simulink model "pgfm_droop"  (R2026b)
settings: Solver=ode1  StartTime=0  StopTime=param.tb.t_end  FixedStep=param.sim.tc
values from neighbouring files (symbols this model uses):
  param = init_pgfm_droop(name)    [pgfm_droop_tests.m]
libraries: fl_lib x52, nesl_utility x6, grid_forming_dqctrl x3
settings Model: Creator=dbagn  LastModifiedBy=dbagn
settings DataIOCC: SaveOutput=off  SaveTime=off  SignalLogging=off
settings SimscapeCC: SimscapeLogType=all  SimscapeNominalValues="[{\"value\":\"1\",\"unit\":\"A\"},{\"value\":\"1\",\"unit\":\"bar\"},{\"value\":\"1\",\"unit\":\"cm^2\"},{\"value\":\"1\",\"unit\":\"cm^3/s\"},{\"value\":\"1\",\"unit\":\"kJ/kg\"},{\"value\":\"1\",\"unit\":\"kW\"},{\"value\":\"1\",\"unit\":\"l\"},{\"value\":\"1\",\"unit\":\"N\"},{\"value\":\"1\",\"unit\":\"N*m\"},{\"value\":\"1\",\"unit\":\"V\"},{\"value\":\"0.001\",\"unit\":\"Wb\"}]"  SimscapeUseEnergyAccounting=off

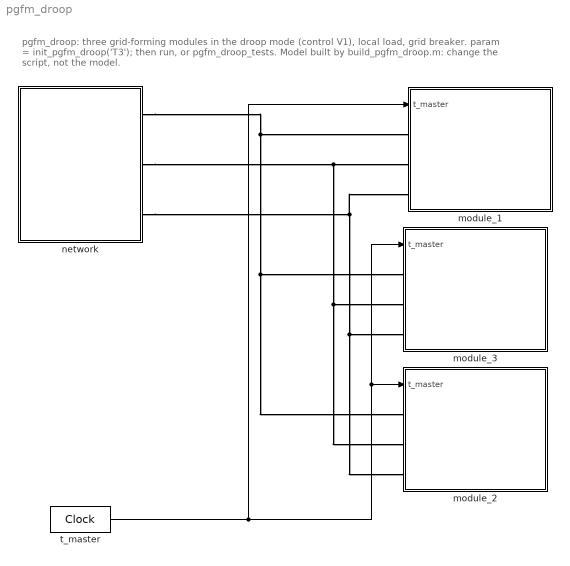
== system pgfm_droop ==
  note: pgfm_droop: three grid-forming modules in the droop mode (control V1), local load, grid breaker.
      | param = init_pgfm_droop('T3'); then run, or pgfm_droop_tests. Model built by build_pgfm_droop.m: change the script, not the model.
  module_1 : Subsystem
  module_2 : Subsystem
  module_3 : Subsystem
  network : Subsystem
  t_master : DigitalClock  SampleTime=param.sim.tc
  wires:
  t_master/1 -> module_1/1(t_master), module_3/1(t_master), module_2/1(t_master)
  connections:
  network/RConn3 -- module_2/LConn3 -- module_3/LConn3 -- module_1/LConn3
  network/RConn1 -- module_2/LConn1 -- module_3/LConn1 -- module_1/LConn1
  network/RConn2 -- module_2/LConn2 -- module_3/LConn2 -- module_1/LConn2

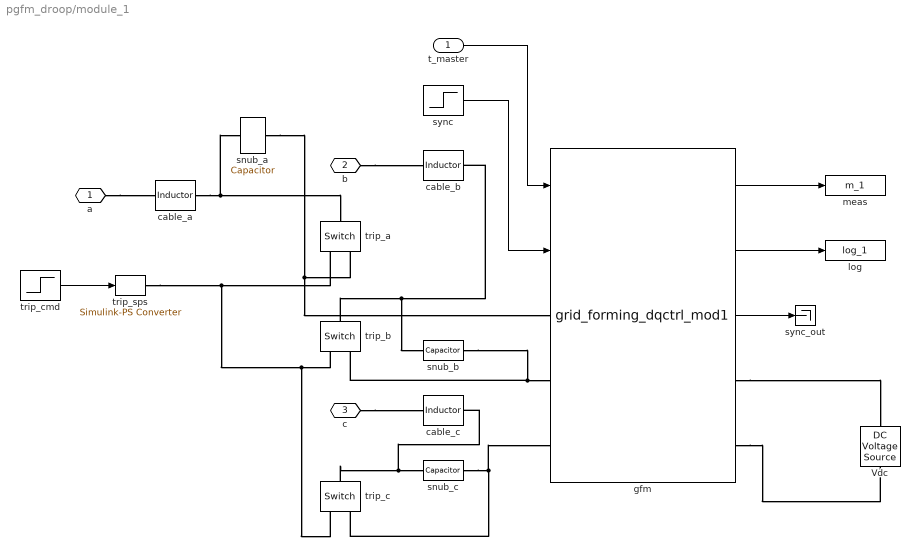
== system pgfm_droop/module_1 ==
  t_master : Inport
  Vdc : fl_lib/Electrical/Electrical Sources/DC Voltage Source  v0=param.mod(1).hw.udc_nom V
  cable_a : fl_lib/Electrical/Electrical Elements/Inductor  l=param.cable.L(1) H  r=param.cable.R(1) Ohm  g=1e-9 1/Ohm  i_specify=off  i_priority=None  i=0 A  i_nominal_specify=off  i_nominal_value=1  i_nominal_unit=A  v_specify=off  v_priority=None  v=0 V  v_nominal_specify=off  v_nominal_value=1  v_nominal_unit=V  i_L_specify=off  i_L_priority=High  i_L=0 A  i_L_nominal_specify=off  i_L_nominal_value=1  i_L_nominal_unit=A
  cable_b : fl_lib/Electrical/Electrical Elements/Inductor  l=param.cable.L(1) H  r=param.cable.R(1) Ohm  g=1e-9 1/Ohm  i_specify=off  i_priority=None  i=0 A  i_nominal_specify=off  i_nominal_value=1  i_nominal_unit=A  v_specify=off  v_priority=None  v=0 V  v_nominal_specify=off  v_nominal_value=1  v_nominal_unit=V  i_L_specify=off  i_L_priority=High  i_L=0 A  i_L_nominal_specify=off  i_L_nominal_value=1  i_L_nominal_unit=A
  cable_c : fl_lib/Electrical/Electrical Elements/Inductor  l=param.cable.L(1) H  r=param.cable.R(1) Ohm  g=1e-9 1/Ohm  i_specify=off  i_priority=None  i=0 A  i_nominal_specify=off  i_nominal_value=1  i_nominal_unit=A  v_specify=off  v_priority=None  v=0 V  v_nominal_specify=off  v_nominal_value=1  v_nominal_unit=V  i_L_specify=off  i_L_priority=High  i_L=0 A  i_L_nominal_specify=off  i_L_nominal_value=1  i_L_nominal_unit=A
  gfm : grid_forming_dqctrl/grid_forming_dqctrl_mod1  p=param.mod(1)
  log : ToWorkspace  VariableName=log_1  SaveFormat=Timeseries  SampleTime=param.sim.ts_log
  meas : ToWorkspace  VariableName=m_1  SaveFormat=Timeseries  SampleTime=param.sim.ts_log
  snub_a : fl_lib/Electrical/Electrical Elements/Capacitor  c=param.snub.C F  r=param.snub.R Ohm  g=0 1/Ohm  i_specify=off  i_priority=None  i=0 A  i_nominal_specify=off  i_nominal_value=1  i_nominal_unit=A  v_specify=off  v_priority=None  v=0 V  v_nominal_specify=off  v_nominal_value=1  v_nominal_unit=V  vc_specify=off  vc_priority=High  vc=0 V  vc_nominal_specify=off  vc_nominal_value=1  vc_nominal_unit=V
  snub_b : fl_lib/Electrical/Electrical Elements/Capacitor  c=param.snub.C F  r=param.snub.R Ohm  g=0 1/Ohm  i_specify=off  i_priority=None  i=0 A  i_nominal_specify=off  i_nominal_value=1  i_nominal_unit=A  v_specify=off  v_priority=None  v=0 V  v_nominal_specify=off  v_nominal_value=1  v_nominal_unit=V  vc_specify=off  vc_priority=High  vc=0 V  vc_nominal_specify=off  vc_nominal_value=1  vc_nominal_unit=V
  snub_c : fl_lib/Electrical/Electrical Elements/Capacitor  c=param.snub.C F  r=param.snub.R Ohm  g=0 1/Ohm  i_specify=off  i_priority=None  i=0 A  i_nominal_specify=off  i_nominal_value=1  i_nominal_unit=A  v_specify=off  v_priority=None  v=0 V  v_nominal_specify=off  v_nominal_value=1  v_nominal_unit=V  vc_specify=off  vc_priority=High  vc=0 V  vc_nominal_specify=off  vc_nominal_value=1  vc_nominal_unit=V
  sync : Step  Time=min(param.tb.sync_t(1), 1e6)  InitialValue=zeros(5, 1)  FinalValue=param.tb.sync_after(:, 1)  SampleTime=param.sim.tc  VectorParams1D=off
  sync_out : Terminator
  trip_a : fl_lib/Electrical/Electrical Elements/Switch  R_closed=1e-4 Ohm  G_open=1e-6 1/Ohm  Threshold=0.5  i_specify=off  i_priority=None  i=0 A  i_nominal_specify=off  i_nominal_value=1  i_nominal_unit=A  v_specify=off  v_priority=None  v=0 V  v_nominal_specify=off  v_nominal_value=1  v_nominal_unit=V
  trip_b : fl_lib/Electrical/Electrical Elements/Switch  R_closed=1e-4 Ohm  G_open=1e-6 1/Ohm  Threshold=0.5  i_specify=off  i_priority=None  i=0 A  i_nominal_specify=off  i_nominal_value=1  i_nominal_unit=A  v_specify=off  v_priority=None  v=0 V  v_nominal_specify=off  v_nominal_value=1  v_nominal_unit=V
  trip_c : fl_lib/Electrical/Electrical Elements/Switch  R_closed=1e-4 Ohm  G_open=1e-6 1/Ohm  Threshold=0.5  i_specify=off  i_priority=None  i=0 A  i_nominal_specify=off  i_nominal_value=1  i_nominal_unit=A  v_specify=off  v_priority=None  v=0 V  v_nominal_specify=off  v_nominal_value=1  v_nominal_unit=V
  trip_cmd : Step  Time=min(param.tb.t_trip(1), 1e6)  InitialValue=1  FinalValue=0  SampleTime=param.sim.tc
  trip_sps : nesl_utility/Simulink-PS Converter  PhysicalDomain=network_engine_domain  SubClassName=ps_input  LeftPortType=input  RightPortType=output  PseudoPeriodic=off  Frequencies=[]  NoiseDistribution=none  NoiseParameters=[]  Unit=1  AffineConversion=off  FilteringAndDerivatives=zero  SimscapeFilterOrder=1  InputFilterTimeConstant=0.001  UdotUserProvided=0
  a : PMIOPort  Side=Left
  b : PMIOPort  Port=2  Side=Left
  c : PMIOPort  Port=3  Side=Left
  wires:
  trip_cmd/1 -> trip_sps/1
  t_master/1 -> gfm/1
  sync/1 -> gfm/2
  gfm/3 -> sync_out/1
  gfm/1 -> meas/1
  gfm/2 -> log/1
  connections:
  trip_sps/RConn1 -- trip_a/RConn1 -- trip_c/RConn1 -- trip_b/RConn1
  gfm/RConn1 -- Vdc/LConn1
  trip_c/LConn1 -- snub_c/LConn1 -- cable_c/RConn1
  a/RConn1 -- cable_a/LConn1
  c/RConn1 -- cable_c/LConn1
  b/RConn1 -- cable_b/LConn1
  cable_a/RConn1 -- trip_a/LConn1 -- snub_a/LConn1
  snub_c/RConn1 -- trip_c/RConn2 -- gfm/LConn3
  snub_a/RConn1 -- trip_a/RConn2 -- gfm/LConn1
  trip_b/LConn1 -- snub_b/LConn1 -- cable_b/RConn1
  snub_b/RConn1 -- trip_b/RConn2 -- gfm/LConn2
  gfm/RConn2 -- Vdc/RConn1

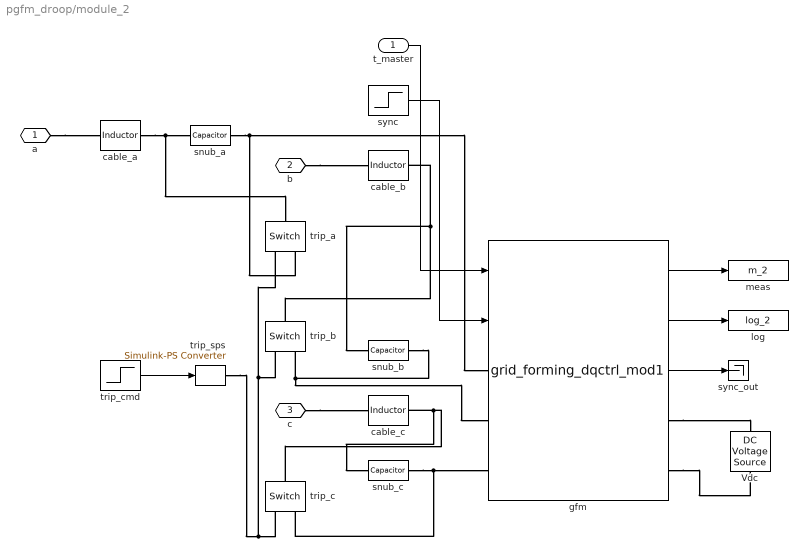
== system pgfm_droop/module_2 ==
  t_master : Inport
  Vdc : fl_lib/Electrical/Electrical Sources/DC Voltage Source  v0=param.mod(2).hw.udc_nom V
  cable_a : fl_lib/Electrical/Electrical Elements/Inductor  l=param.cable.L(2) H  r=param.cable.R(2) Ohm  g=1e-9 1/Ohm  i_specify=off  i_priority=None  i=0 A  i_nominal_specify=off  i_nominal_value=1  i_nominal_unit=A  v_specify=off  v_priority=None  v=0 V  v_nominal_specify=off  v_nominal_value=1  v_nominal_unit=V  i_L_specify=off  i_L_priority=High  i_L=0 A  i_L_nominal_specify=off  i_L_nominal_value=1  i_L_nominal_unit=A
  cable_b : fl_lib/Electrical/Electrical Elements/Inductor  l=param.cable.L(2) H  r=param.cable.R(2) Ohm  g=1e-9 1/Ohm  i_specify=off  i_priority=None  i=0 A  i_nominal_specify=off  i_nominal_value=1  i_nominal_unit=A  v_specify=off  v_priority=None  v=0 V  v_nominal_specify=off  v_nominal_value=1  v_nominal_unit=V  i_L_specify=off  i_L_priority=High  i_L=0 A  i_L_nominal_specify=off  i_L_nominal_value=1  i_L_nominal_unit=A
  cable_c : fl_lib/Electrical/Electrical Elements/Inductor  l=param.cable.L(2) H  r=param.cable.R(2) Ohm  g=1e-9 1/Ohm  i_specify=off  i_priority=None  i=0 A  i_nominal_specify=off  i_nominal_value=1  i_nominal_unit=A  v_specify=off  v_priority=None  v=0 V  v_nominal_specify=off  v_nominal_value=1  v_nominal_unit=V  i_L_specify=off  i_L_priority=High  i_L=0 A  i_L_nominal_specify=off  i_L_nominal_value=1  i_L_nominal_unit=A
  gfm : grid_forming_dqctrl/grid_forming_dqctrl_mod1  p=param.mod(2)
  log : ToWorkspace  VariableName=log_2  SaveFormat=Timeseries  SampleTime=param.sim.ts_log
  meas : ToWorkspace  VariableName=m_2  SaveFormat=Timeseries  SampleTime=param.sim.ts_log
  snub_a : fl_lib/Electrical/Electrical Elements/Capacitor  c=param.snub.C F  r=param.snub.R Ohm  g=0 1/Ohm  i_specify=off  i_priority=None  i=0 A  i_nominal_specify=off  i_nominal_value=1  i_nominal_unit=A  v_specify=off  v_priority=None  v=0 V  v_nominal_specify=off  v_nominal_value=1  v_nominal_unit=V  vc_specify=off  vc_priority=High  vc=0 V  vc_nominal_specify=off  vc_nominal_value=1  vc_nominal_unit=V
  snub_b : fl_lib/Electrical/Electrical Elements/Capacitor  c=param.snub.C F  r=param.snub.R Ohm  g=0 1/Ohm  i_specify=off  i_priority=None  i=0 A  i_nominal_specify=off  i_nominal_value=1  i_nominal_unit=A  v_specify=off  v_priority=None  v=0 V  v_nominal_specify=off  v_nominal_value=1  v_nominal_unit=V  vc_specify=off  vc_priority=High  vc=0 V  vc_nominal_specify=off  vc_nominal_value=1  vc_nominal_unit=V
  snub_c : fl_lib/Electrical/Electrical Elements/Capacitor  c=param.snub.C F  r=param.snub.R Ohm  g=0 1/Ohm  i_specify=off  i_priority=None  i=0 A  i_nominal_specify=off  i_nominal_value=1  i_nominal_unit=A  v_specify=off  v_priority=None  v=0 V  v_nominal_specify=off  v_nominal_value=1  v_nominal_unit=V  vc_specify=off  vc_priority=High  vc=0 V  vc_nominal_specify=off  vc_nominal_value=1  vc_nominal_unit=V
  sync : Step  Time=min(param.tb.sync_t(2), 1e6)  InitialValue=zeros(5, 1)  FinalValue=param.tb.sync_after(:, 2)  SampleTime=param.sim.tc  VectorParams1D=off
  sync_out : Terminator
  trip_a : fl_lib/Electrical/Electrical Elements/Switch  R_closed=1e-4 Ohm  G_open=1e-6 1/Ohm  Threshold=0.5  i_specify=off  i_priority=None  i=0 A  i_nominal_specify=off  i_nominal_value=1  i_nominal_unit=A  v_specify=off  v_priority=None  v=0 V  v_nominal_specify=off  v_nominal_value=1  v_nominal_unit=V
  trip_b : fl_lib/Electrical/Electrical Elements/Switch  R_closed=1e-4 Ohm  G_open=1e-6 1/Ohm  Threshold=0.5  i_specify=off  i_priority=None  i=0 A  i_nominal_specify=off  i_nominal_value=1  i_nominal_unit=A  v_specify=off  v_priority=None  v=0 V  v_nominal_specify=off  v_nominal_value=1  v_nominal_unit=V
  trip_c : fl_lib/Electrical/Electrical Elements/Switch  R_closed=1e-4 Ohm  G_open=1e-6 1/Ohm  Threshold=0.5  i_specify=off  i_priority=None  i=0 A  i_nominal_specify=off  i_nominal_value=1  i_nominal_unit=A  v_specify=off  v_priority=None  v=0 V  v_nominal_specify=off  v_nominal_value=1  v_nominal_unit=V
  trip_cmd : Step  Time=min(param.tb.t_trip(2), 1e6)  InitialValue=1  FinalValue=0  SampleTime=param.sim.tc
  trip_sps : nesl_utility/Simulink-PS Converter  PhysicalDomain=network_engine_domain  SubClassName=ps_input  LeftPortType=input  RightPortType=output  PseudoPeriodic=off  Frequencies=[]  NoiseDistribution=none  NoiseParameters=[]  Unit=1  AffineConversion=off  FilteringAndDerivatives=zero  SimscapeFilterOrder=1  InputFilterTimeConstant=0.001  UdotUserProvided=0
  a : PMIOPort  Side=Left
  b : PMIOPort  Port=2  Side=Left
  c : PMIOPort  Port=3  Side=Left
  wires:
  trip_cmd/1 -> trip_sps/1
  sync/1 -> gfm/2
  t_master/1 -> gfm/1
  gfm/1 -> meas/1
  gfm/2 -> log/1
  gfm/3 -> sync_out/1
  connections:
  a/RConn1 -- cable_a/LConn1
  c/RConn1 -- cable_c/LConn1
  trip_sps/RConn1 -- trip_b/RConn1 -- trip_a/RConn1 -- trip_c/RConn1
  b/RConn1 -- cable_b/LConn1
  cable_a/RConn1 -- trip_a/LConn1 -- snub_a/LConn1
  gfm/RConn1 -- Vdc/LConn1
  snub_a/RConn1 -- gfm/LConn1 -- trip_a/RConn2
  trip_c/LConn1 -- cable_c/RConn1 -- snub_c/LConn1
  trip_b/LConn1 -- cable_b/RConn1 -- snub_b/LConn1
  snub_b/RConn1 -- trip_b/RConn2 -- gfm/LConn2
  snub_c/RConn1 -- trip_c/RConn2 -- gfm/LConn3
  gfm/RConn2 -- Vdc/RConn1

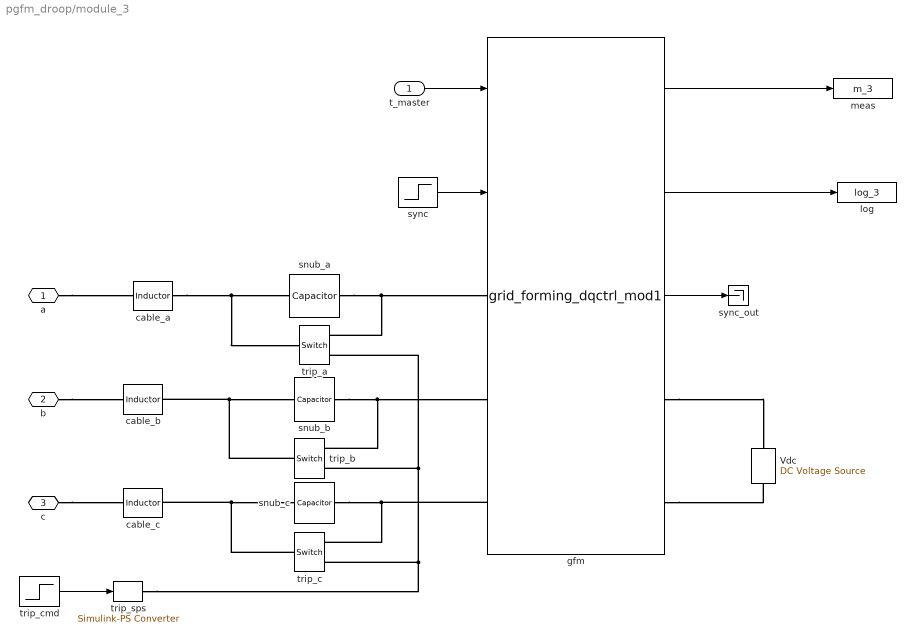
== system pgfm_droop/module_3 ==
  t_master : Inport
  Vdc : fl_lib/Electrical/Electrical Sources/DC Voltage Source  v0=param.mod(3).hw.udc_nom V
  cable_a : fl_lib/Electrical/Electrical Elements/Inductor  l=param.cable.L(3) H  r=param.cable.R(3) Ohm  g=1e-9 1/Ohm  i_specify=off  i_priority=None  i=0 A  i_nominal_specify=off  i_nominal_value=1  i_nominal_unit=A  v_specify=off  v_priority=None  v=0 V  v_nominal_specify=off  v_nominal_value=1  v_nominal_unit=V  i_L_specify=off  i_L_priority=High  i_L=0 A  i_L_nominal_specify=off  i_L_nominal_value=1  i_L_nominal_unit=A
  cable_b : fl_lib/Electrical/Electrical Elements/Inductor  l=param.cable.L(3) H  r=param.cable.R(3) Ohm  g=1e-9 1/Ohm  i_specify=off  i_priority=None  i=0 A  i_nominal_specify=off  i_nominal_value=1  i_nominal_unit=A  v_specify=off  v_priority=None  v=0 V  v_nominal_specify=off  v_nominal_value=1  v_nominal_unit=V  i_L_specify=off  i_L_priority=High  i_L=0 A  i_L_nominal_specify=off  i_L_nominal_value=1  i_L_nominal_unit=A
  cable_c : fl_lib/Electrical/Electrical Elements/Inductor  l=param.cable.L(3) H  r=param.cable.R(3) Ohm  g=1e-9 1/Ohm  i_specify=off  i_priority=None  i=0 A  i_nominal_specify=off  i_nominal_value=1  i_nominal_unit=A  v_specify=off  v_priority=None  v=0 V  v_nominal_specify=off  v_nominal_value=1  v_nominal_unit=V  i_L_specify=off  i_L_priority=High  i_L=0 A  i_L_nominal_specify=off  i_L_nominal_value=1  i_L_nominal_unit=A
  gfm : grid_forming_dqctrl/grid_forming_dqctrl_mod1  p=param.mod(3)
  log : ToWorkspace  VariableName=log_3  SaveFormat=Timeseries  SampleTime=param.sim.ts_log
  meas : ToWorkspace  VariableName=m_3  SaveFormat=Timeseries  SampleTime=param.sim.ts_log
  snub_a : fl_lib/Electrical/Electrical Elements/Capacitor  c=param.snub.C F  r=param.snub.R Ohm  g=0 1/Ohm  i_specify=off  i_priority=None  i=0 A  i_nominal_specify=off  i_nominal_value=1  i_nominal_unit=A  v_specify=off  v_priority=None  v=0 V  v_nominal_specify=off  v_nominal_value=1  v_nominal_unit=V  vc_specify=off  vc_priority=High  vc=0 V  vc_nominal_specify=off  vc_nominal_value=1  vc_nominal_unit=V
  snub_b : fl_lib/Electrical/Electrical Elements/Capacitor  c=param.snub.C F  r=param.snub.R Ohm  g=0 1/Ohm  i_specify=off  i_priority=None  i=0 A  i_nominal_specify=off  i_nominal_value=1  i_nominal_unit=A  v_specify=off  v_priority=None  v=0 V  v_nominal_specify=off  v_nominal_value=1  v_nominal_unit=V  vc_specify=off  vc_priority=High  vc=0 V  vc_nominal_specify=off  vc_nominal_value=1  vc_nominal_unit=V
  snub_c : fl_lib/Electrical/Electrical Elements/Capacitor  c=param.snub.C F  r=param.snub.R Ohm  g=0 1/Ohm  i_specify=off  i_priority=None  i=0 A  i_nominal_specify=off  i_nominal_value=1  i_nominal_unit=A  v_specify=off  v_priority=None  v=0 V  v_nominal_specify=off  v_nominal_value=1  v_nominal_unit=V  vc_specify=off  vc_priority=High  vc=0 V  vc_nominal_specify=off  vc_nominal_value=1  vc_nominal_unit=V
  sync : Step  Time=min(param.tb.sync_t(3), 1e6)  InitialValue=zeros(5, 1)  FinalValue=param.tb.sync_after(:, 3)  SampleTime=param.sim.tc  VectorParams1D=off
  sync_out : Terminator
  trip_a : fl_lib/Electrical/Electrical Elements/Switch  R_closed=1e-4 Ohm  G_open=1e-6 1/Ohm  Threshold=0.5  i_specify=off  i_priority=None  i=0 A  i_nominal_specify=off  i_nominal_value=1  i_nominal_unit=A  v_specify=off  v_priority=None  v=0 V  v_nominal_specify=off  v_nominal_value=1  v_nominal_unit=V
  trip_b : fl_lib/Electrical/Electrical Elements/Switch  R_closed=1e-4 Ohm  G_open=1e-6 1/Ohm  Threshold=0.5  i_specify=off  i_priority=None  i=0 A  i_nominal_specify=off  i_nominal_value=1  i_nominal_unit=A  v_specify=off  v_priority=None  v=0 V  v_nominal_specify=off  v_nominal_value=1  v_nominal_unit=V
  trip_c : fl_lib/Electrical/Electrical Elements/Switch  R_closed=1e-4 Ohm  G_open=1e-6 1/Ohm  Threshold=0.5  i_specify=off  i_priority=None  i=0 A  i_nominal_specify=off  i_nominal_value=1  i_nominal_unit=A  v_specify=off  v_priority=None  v=0 V  v_nominal_specify=off  v_nominal_value=1  v_nominal_unit=V
  trip_cmd : Step  Time=min(param.tb.t_trip(3), 1e6)  InitialValue=1  FinalValue=0  SampleTime=param.sim.tc
  trip_sps : nesl_utility/Simulink-PS Converter  PhysicalDomain=network_engine_domain  SubClassName=ps_input  LeftPortType=input  RightPortType=output  PseudoPeriodic=off  Frequencies=[]  NoiseDistribution=none  NoiseParameters=[]  Unit=1  AffineConversion=off  FilteringAndDerivatives=zero  SimscapeFilterOrder=1  InputFilterTimeConstant=0.001  UdotUserProvided=0
  a : PMIOPort  Side=Left
  b : PMIOPort  Port=2  Side=Left
  c : PMIOPort  Port=3  Side=Left
  wires:
  gfm/3 -> sync_out/1
  sync/1 -> gfm/2
  trip_cmd/1 -> trip_sps/1
  t_master/1 -> gfm/1
  gfm/2 -> log/1
  gfm/1 -> meas/1
  connections:
  trip_c/LConn1 -- cable_c/RConn1 -- snub_c/LConn1
  snub_a/RConn1 -- gfm/LConn1 -- trip_a/RConn2
  trip_b/LConn1 -- cable_b/RConn1 -- snub_b/LConn1
  gfm/RConn1 -- Vdc/LConn1
  b/RConn1 -- cable_b/LConn1
  c/RConn1 -- cable_c/LConn1
  trip_sps/RConn1 -- trip_c/RConn1 -- trip_b/RConn1 -- trip_a/RConn1
  a/RConn1 -- cable_a/LConn1
  cable_a/RConn1 -- snub_a/LConn1 -- trip_a/LConn1
  snub_b/RConn1 -- gfm/LConn2 -- trip_b/RConn2
  gfm/LConn3 -- snub_c/RConn1 -- trip_c/RConn2
  gfm/RConn2 -- Vdc/RConn1

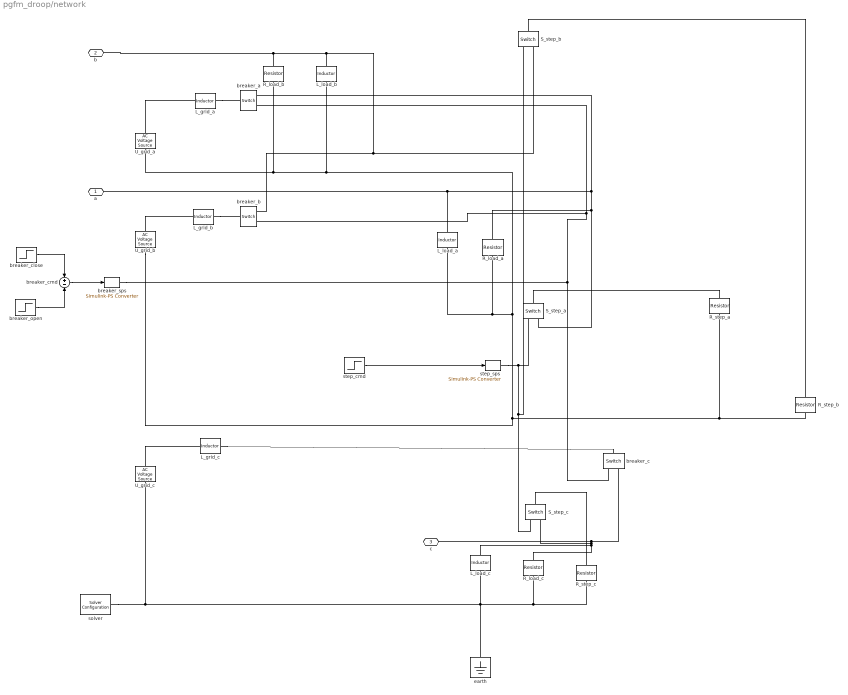
== system pgfm_droop/network ==
  L_grid_a : fl_lib/Electrical/Electrical Elements/Inductor  l=param.grid.L H  r=param.grid.R Ohm  g=1e-9 1/Ohm  i_specify=off  i_priority=None  i=0 A  i_nominal_specify=off  i_nominal_value=1  i_nominal_unit=A  v_specify=off  v_priority=None  v=0 V  v_nominal_specify=off  v_nominal_value=1  v_nominal_unit=V  i_L_specify=off  i_L_priority=High  i_L=0 A  i_L_nominal_specify=off  i_L_nominal_value=1  i_L_nominal_unit=A
  L_grid_b : fl_lib/Electrical/Electrical Elements/Inductor  l=param.grid.L H  r=param.grid.R Ohm  g=1e-9 1/Ohm  i_specify=off  i_priority=None  i=0 A  i_nominal_specify=off  i_nominal_value=1  i_nominal_unit=A  v_specify=off  v_priority=None  v=0 V  v_nominal_specify=off  v_nominal_value=1  v_nominal_unit=V  i_L_specify=off  i_L_priority=High  i_L=0 A  i_L_nominal_specify=off  i_L_nominal_value=1  i_L_nominal_unit=A
  L_grid_c : fl_lib/Electrical/Electrical Elements/Inductor  l=param.grid.L H  r=param.grid.R Ohm  g=1e-9 1/Ohm  i_specify=off  i_priority=None  i=0 A  i_nominal_specify=off  i_nominal_value=1  i_nominal_unit=A  v_specify=off  v_priority=None  v=0 V  v_nominal_specify=off  v_nominal_value=1  v_nominal_unit=V  i_L_specify=off  i_L_priority=High  i_L=0 A  i_L_nominal_specify=off  i_L_nominal_value=1  i_L_nominal_unit=A
  L_load_a : fl_lib/Electrical/Electrical Elements/Inductor  l=param.load.L H  r=param.load.RL Ohm  g=1e-9 1/Ohm  i_specify=off  i_priority=None  i=0 A  i_nominal_specify=off  i_nominal_value=1  i_nominal_unit=A  v_specify=off  v_priority=None  v=0 V  v_nominal_specify=off  v_nominal_value=1  v_nominal_unit=V  i_L_specify=off  i_L_priority=High  i_L=0 A  i_L_nominal_specify=off  i_L_nominal_value=1  i_L_nominal_unit=A
  L_load_b : fl_lib/Electrical/Electrical Elements/Inductor  l=param.load.L H  r=param.load.RL Ohm  g=1e-9 1/Ohm  i_specify=off  i_priority=None  i=0 A  i_nominal_specify=off  i_nominal_value=1  i_nominal_unit=A  v_specify=off  v_priority=None  v=0 V  v_nominal_specify=off  v_nominal_value=1  v_nominal_unit=V  i_L_specify=off  i_L_priority=High  i_L=0 A  i_L_nominal_specify=off  i_L_nominal_value=1  i_L_nominal_unit=A
  L_load_c : fl_lib/Electrical/Electrical Elements/Inductor  l=param.load.L H  r=param.load.RL Ohm  g=1e-9 1/Ohm  i_specify=off  i_priority=None  i=0 A  i_nominal_specify=off  i_nominal_value=1  i_nominal_unit=A  v_specify=off  v_priority=None  v=0 V  v_nominal_specify=off  v_nominal_value=1  v_nominal_unit=V  i_L_specify=off  i_L_priority=High  i_L=0 A  i_L_nominal_specify=off  i_L_nominal_value=1  i_L_nominal_unit=A
  R_load_a : fl_lib/Electrical/Electrical Elements/Resistor  R=param.load.R Ohm  i_specify=off  i_priority=None  i=0 A  i_nominal_specify=off  i_nominal_value=1  i_nominal_unit=A  v_specify=off  v_priority=None  v=0 V  v_nominal_specify=off  v_nominal_value=1  v_nominal_unit=V
  R_load_b : fl_lib/Electrical/Electrical Elements/Resistor  R=param.load.R Ohm  i_specify=off  i_priority=None  i=0 A  i_nominal_specify=off  i_nominal_value=1  i_nominal_unit=A  v_specify=off  v_priority=None  v=0 V  v_nominal_specify=off  v_nominal_value=1  v_nominal_unit=V
  R_load_c : fl_lib/Electrical/Electrical Elements/Resistor  R=param.load.R Ohm  i_specify=off  i_priority=None  i=0 A  i_nominal_specify=off  i_nominal_value=1  i_nominal_unit=A  v_specify=off  v_priority=None  v=0 V  v_nominal_specify=off  v_nominal_value=1  v_nominal_unit=V
  R_step_a : fl_lib/Electrical/Electrical Elements/Resistor  R=param.load.R_step Ohm  i_specify=off  i_priority=None  i=0 A  i_nominal_specify=off  i_nominal_value=1  i_nominal_unit=A  v_specify=off  v_priority=None  v=0 V  v_nominal_specify=off  v_nominal_value=1  v_nominal_unit=V
  R_step_b : fl_lib/Electrical/Electrical Elements/Resistor  R=param.load.R_step Ohm  i_specify=off  i_priority=None  i=0 A  i_nominal_specify=off  i_nominal_value=1  i_nominal_unit=A  v_specify=off  v_priority=None  v=0 V  v_nominal_specify=off  v_nominal_value=1  v_nominal_unit=V
  R_step_c : fl_lib/Electrical/Electrical Elements/Resistor  R=param.load.R_step Ohm  i_specify=off  i_priority=None  i=0 A  i_nominal_specify=off  i_nominal_value=1  i_nominal_unit=A  v_specify=off  v_priority=None  v=0 V  v_nominal_specify=off  v_nominal_value=1  v_nominal_unit=V
  S_step_a : fl_lib/Electrical/Electrical Elements/Switch  R_closed=1e-4 Ohm  G_open=1e-6 1/Ohm  Threshold=0.5  i_specify=off  i_priority=None  i=0 A  i_nominal_specify=off  i_nominal_value=1  i_nominal_unit=A  v_specify=off  v_priority=None  v=0 V  v_nominal_specify=off  v_nominal_value=1  v_nominal_unit=V
  S_step_b : fl_lib/Electrical/Electrical Elements/Switch  R_closed=1e-4 Ohm  G_open=1e-6 1/Ohm  Threshold=0.5  i_specify=off  i_priority=None  i=0 A  i_nominal_specify=off  i_nominal_value=1  i_nominal_unit=A  v_specify=off  v_priority=None  v=0 V  v_nominal_specify=off  v_nominal_value=1  v_nominal_unit=V
  S_step_c : fl_lib/Electrical/Electrical Elements/Switch  R_closed=1e-4 Ohm  G_open=1e-6 1/Ohm  Threshold=0.5  i_specify=off  i_priority=None  i=0 A  i_nominal_specify=off  i_nominal_value=1  i_nominal_unit=A  v_specify=off  v_priority=None  v=0 V  v_nominal_specify=off  v_nominal_value=1  v_nominal_unit=V
  U_grid_a : fl_lib/Electrical/Electrical Sources/AC Voltage Source  amp=param.grid.u_peak V  shift=0 deg  frequency=param.grid.f Hz
  U_grid_b : fl_lib/Electrical/Electrical Sources/AC Voltage Source  amp=param.grid.u_peak V  shift=-120 deg  frequency=param.grid.f Hz
  U_grid_c : fl_lib/Electrical/Electrical Sources/AC Voltage Source  amp=param.grid.u_peak V  shift=120 deg  frequency=param.grid.f Hz
  breaker_a : fl_lib/Electrical/Electrical Elements/Switch  R_closed=1e-4 Ohm  G_open=1e-6 1/Ohm  Threshold=0.5  i_specify=off  i_priority=None  i=0 A  i_nominal_specify=off  i_nominal_value=1  i_nominal_unit=A  v_specify=off  v_priority=None  v=0 V  v_nominal_specify=off  v_nominal_value=1  v_nominal_unit=V
  breaker_b : fl_lib/Electrical/Electrical Elements/Switch  R_closed=1e-4 Ohm  G_open=1e-6 1/Ohm  Threshold=0.5  i_specify=off  i_priority=None  i=0 A  i_nominal_specify=off  i_nominal_value=1  i_nominal_unit=A  v_specify=off  v_priority=None  v=0 V  v_nominal_specify=off  v_nominal_value=1  v_nominal_unit=V
  breaker_c : fl_lib/Electrical/Electrical Elements/Switch  R_closed=1e-4 Ohm  G_open=1e-6 1/Ohm  Threshold=0.5  i_specify=off  i_priority=None  i=0 A  i_nominal_specify=off  i_nominal_value=1  i_nominal_unit=A  v_specify=off  v_priority=None  v=0 V  v_nominal_specify=off  v_nominal_value=1  v_nominal_unit=V
  breaker_close : Step  Time=min(param.tb.t_close, 1e6)  SampleTime=param.sim.tc
  breaker_cmd : Sum  Inputs=+-
  breaker_open : Step  Time=min(param.tb.t_open, 1e6)  SampleTime=param.sim.tc
  breaker_sps : nesl_utility/Simulink-PS Converter  PhysicalDomain=network_engine_domain  SubClassName=ps_input  LeftPortType=input  RightPortType=output  PseudoPeriodic=off  Frequencies=[]  NoiseDistribution=none  NoiseParameters=[]  Unit=1  AffineConversion=off  FilteringAndDerivatives=zero  SimscapeFilterOrder=1  InputFilterTimeConstant=0.001  UdotUserProvided=0
  earth : fl_lib/Electrical/Electrical Elements/Electrical Reference
  solver : nesl_utility/Solver Configuration  PhysicalDomain=network_engine_domain  SubClassName=solver  LeftPortType=input  RightPortType=generic  Tones=[]  Harmonics=[]  SimulateNoise=off  Profile=off  UseLocalSampling=off  EnableSwitchedLinearOptims=on  FrequencyDomain=off  UseCCode=off  RelTol=0.001  AbsTol=0.001  MinStep=1e-09  ToWorkspace=off  RevertToSquareIcSolve=off  NumHomotopyIterations=100  PhasorMode=off  PhasorModeNumHarmonics=1  ConsistencySolver=NEWTON_XTOL_AFTER_FTOL  CanonicalOrdering=CANONICAL  OptimizeIntermediates=OPTIMIZED  MulticoreSolverChoice=BACKWARD_EULER  IndexReductionMethod=DerivativeReplacement  DoDC=on  ResidualTolerance=1e-09  ConsistencyTolSource=GLOBAL  ConsistencyAbsTol=0.001  ConsistencyRelTol=0.001  ConsistencyTolFactor=0.001  UseLocalSolver=on  LocalSolverChoice=NE_BACKWARD_EULER_ADVANCER  ResolveIndetEquations=on  FunctionEvalNumThread=1  LocalSolverSampleTime=param.sim.tc  DoFixedCost=on  MaxNonlinIter=param.sim.nonlinear_iterations  MaxModeIter=2  ComputeImpulses=off  ImpulseIterations=2  LinearAlgebra=auto  LinearAlgebraNumThread=0  EquationFormulation=NE_TIME_EF  DelaysMemoryBudget=1024  AutomaticFiltering=on  FilteringTimeConstant=0.001  PartitionStorageMethod=AS_NEEDED  PartitionMemoryBudget=1024  PartitionMethod=BALANCED  MultibodyUseLocalSolver=off  MultibodyLocalSolverChoice=ODE1  MultibodyLocalSolverSampleTime=0.001
  step_cmd : Step  Time=min(param.tb.t_step, 1e6)  SampleTime=param.sim.tc
  step_sps : nesl_utility/Simulink-PS Converter  PhysicalDomain=network_engine_domain  SubClassName=ps_input  LeftPortType=input  RightPortType=output  PseudoPeriodic=off  Frequencies=[]  NoiseDistribution=none  NoiseParameters=[]  Unit=1  AffineConversion=off  FilteringAndDerivatives=zero  SimscapeFilterOrder=1  InputFilterTimeConstant=0.001  UdotUserProvided=0
  a : PMIOPort  Side=Right
  b : PMIOPort  Port=2  Side=Right
  c : PMIOPort  Port=3  Side=Right
  wires:
  step_cmd/1 -> step_sps/1
  breaker_open/1 -> breaker_cmd/2
  breaker_close/1 -> breaker_cmd/1
  breaker_cmd/1 -> breaker_sps/1
  connections:
  U_grid_a/LConn1 -- L_grid_a/LConn1
  solver/RConn1 -- L_load_c/RConn1 -- R_load_c/RConn1 -- R_step_c/RConn1 -- earth/LConn1 -- U_grid_c/RConn1
  U_grid_b/RConn1 -- U_grid_a/RConn1 -- R_load_b/RConn1 -- L_load_b/RConn1 -- R_load_a/RConn1 -- L_load_a/RConn1 -- R_step_b/RConn1 -- R_step_a/RConn1
  U_grid_b/LConn1 -- L_grid_b/LConn1
  S_step_a/LConn1 -- R_step_a/LConn1
  L_grid_b/RConn1 -- breaker_b/LConn1
  R_load_b/LConn1 -- S_step_b/RConn2 -- breaker_b/RConn2 -- L_load_b/LConn1 -- b/RConn1
  L_load_a/LConn1 -- R_load_a/LConn1 -- S_step_a/RConn2 -- breaker_a/RConn2 -- a/RConn1
  step_sps/RConn1 -- S_step_c/RConn1 -- S_step_b/RConn1 -- S_step_a/RConn1
  U_grid_c/LConn1 -- L_grid_c/LConn1
  L_load_c/LConn1 -- breaker_c/RConn2 -- c/RConn1 -- S_step_c/RConn2 -- R_load_c/LConn1
  L_grid_a/RConn1 -- breaker_a/LConn1
  breaker_sps/RConn1 -- breaker_a/RConn1 -- breaker_b/RConn1 -- breaker_c/RConn1
  S_step_b/LConn1 -- R_step_b/LConn1
  L_grid_c/RConn1 -- breaker_c/LConn1
  S_step_c/LConn1 -- R_step_c/LConn1
